simulink model "carpark_shuffler_sim"  (R2025b)
settings: Solver=VariableStepAuto  StartTime=0.0  StopTime=0.06  MaxStep=1e-4  RelTol=1e-4
PreLoadFcn:
  | init_params;
InitFcn:
  | init_params
undefined symbols (not defined in the file or in its folder): LOADP, SENSE, SRC
libraries: fl_lib x63, ee_lib x43, nesl_utility x37
(part 1 of 4)
settings Model: SimulationMode=accelerator  Creator=jazsa  LastModifiedBy=jazsa
settings SolverCC: ZeroCrossAlgorithm=Adaptive
settings DataIOCC: SignalLogging=off

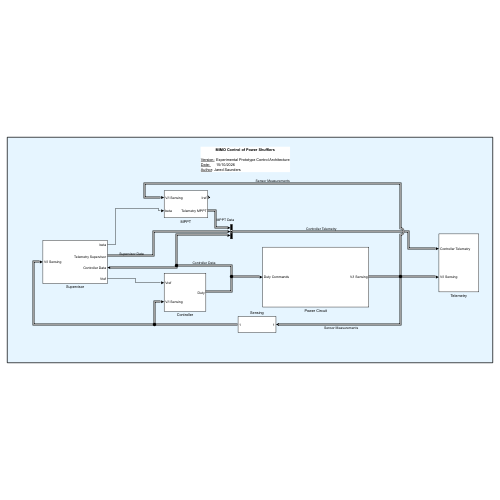
[thumbnail: Simulink's stored preview of the top-level diagram]
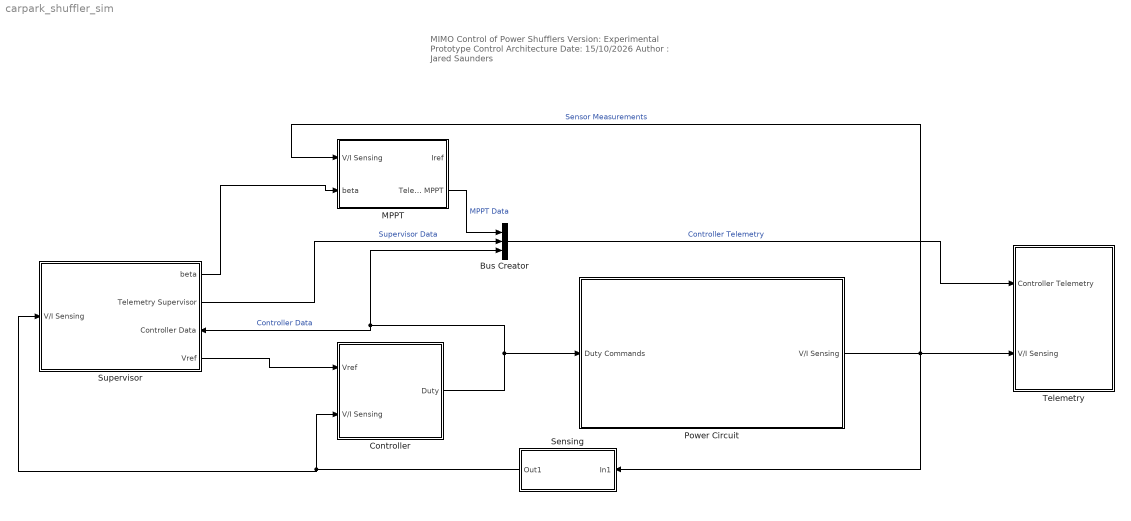
== system carpark_shuffler_sim ==
  note: MIMO Control of Power Shufflers
      |
      | Version: Experimental Prototype Control Architecture
      | Date: 15/10/2026
      | Author : Jared Saunders
  Bus Creator : BusCreator  Inputs=3
  Controller : Subsystem
  MPPT : Subsystem
  Power Circuit : Subsystem
  Sensing : Subsystem
  Supervisor : Subsystem
      settings: PortSchema="{\"entries\":[{\"content\":{\"sides\":[{\"content\":{\"connectorIds\":[\"In1\"]},\"type\":\"ConnectorPlacement.EquallySpacedRectSide\",\"uuid\":\"4149ece3-2139-4a6b-be3b-85e3b5016338\"},{\"content\":{\"connectorIds\":[\"Out1\",\"Out2\",\"In2\",\"Out3\"],\"side\":\"RIGHT\"},\"type\":\"ConnectorPlacement.EquallySpacedRectSide\",\"uuid\":\"a4c8f16e-63c5-4e73-b921-9be0544bd052\"},{\"content\":{\"side\":\"TOP\"},\"type\":\"ConnectorPlacement.EquallySpacedRectSide\",\"uuid\":\"efcb0ad6-b028-42ed-a2aa-71b179d48e39\"}]},\"type\":\"ConnectorPlacement.EquallySpacedConnector\",\"uuid\":\"3400d1fe-81e3-4212-a4bc-db484173b6e0\"}],\"packageUris\":[\"http://schema.mathworks.com/mf0/Connector/R2020b\"],\"version\":\"1.0\"}"
  Telemetry : Subsystem
  wires:
  Supervisor/1(beta) -> MPPT/2(beta)
  Power Circuit/1(V/I Sensing) -> MPPT/1(V/I Sensing), Telemetry/2(V/I Sensing), Sensing/1(In1)  "Sensor Measurements"
  Supervisor/3(Vref) -> Controller/1(Vref)
  Controller/1(Duty) -> Power Circuit/1(Duty Commands), Bus Creator/3, Supervisor/2(Controller Data)  "Controller Data"
  MPPT/2(Telemetry MPPT) -> Bus Creator/1  "MPPT Data"
  Supervisor/2(Telemetry Supervisor) -> Bus Creator/2  "Supervisor Data"
  Bus Creator/1 -> Telemetry/1(Controller Telemetry)  "Controller Telemetry"
  Sensing/1(Out1) -> Supervisor/1(V/I Sensing), Controller/2(V/I Sensing)

== system carpark_shuffler_sim/Controller ==
  Vref : Inport
  V/I Sensing : Inport  Port=2
  Bus Creator : BusCreator  Inputs=4
  Bus Selector : BusSelector  OutputSignals=Module Voltages,Phase Currents
  Controller : MATLAB Function  TreatAsAtomicUnit=on  SystemSampleTime=100e-6
  Demux : Demux
  Duty : Outport
  wires:
  Bus Selector/1 -> Controller/1(VM)  "<Module Voltages>"
  V/I Sensing/1 -> Bus Selector/1
  Bus Selector/2 -> Controller/2(IL)  "<Phase Currents>"
  Vref/1 -> Controller/3(rv)
  Controller/1(d) -> Demux/1
  Demux/1 -> Bus Creator/1  "dA1"
  Demux/2 -> Bus Creator/2  "dB1"
  Demux/3 -> Bus Creator/3  "dA2"
  Demux/4 -> Bus Creator/4  "dB2"
  Bus Creator/1 -> Duty/1

== system carpark_shuffler_sim/MPPT ==
  V/I Sensing : Inport
  beta : Inport  Port=2
  Bus Creator : BusCreator  Inputs=3
  Bus Selector : BusSelector  OutputSignals=String Power Meter
  Bus Selector1 : BusSelector  OutputSignals=V_string,I_string
  Delay : UnitDelay  InitialCondition=12  SampleTime=1e-3  HasFrameUpgradeWarning=on
  Enable : Constant  Value=0
  P&O : MATLAB Function  TreatAsAtomicUnit=on  SystemSampleTime=1e-3
  Iref : Outport
  Telemetry MPPT : Outport  Port=2
  wires:
  beta/1 -> P&O/3(beta)
  V/I Sensing/1 -> Bus Selector/1
  P&O/3(state) -> Bus Creator/3
  Bus Selector1/1 -> P&O/1(Vstr)  "<V_string>"
  Bus Selector1/2 -> P&O/2(Istr)  "<I_string>"
  P&O/1(Iref) -> Bus Creator/1, Delay/1
  Delay/1 -> Iref/1
  Enable/1 -> P&O/4(en)
  Bus Creator/1 -> Telemetry MPPT/1
  P&O/2(Pav) -> Bus Creator/2
  Bus Selector/1 -> Bus Selector1/1  "<String Power Meter>"

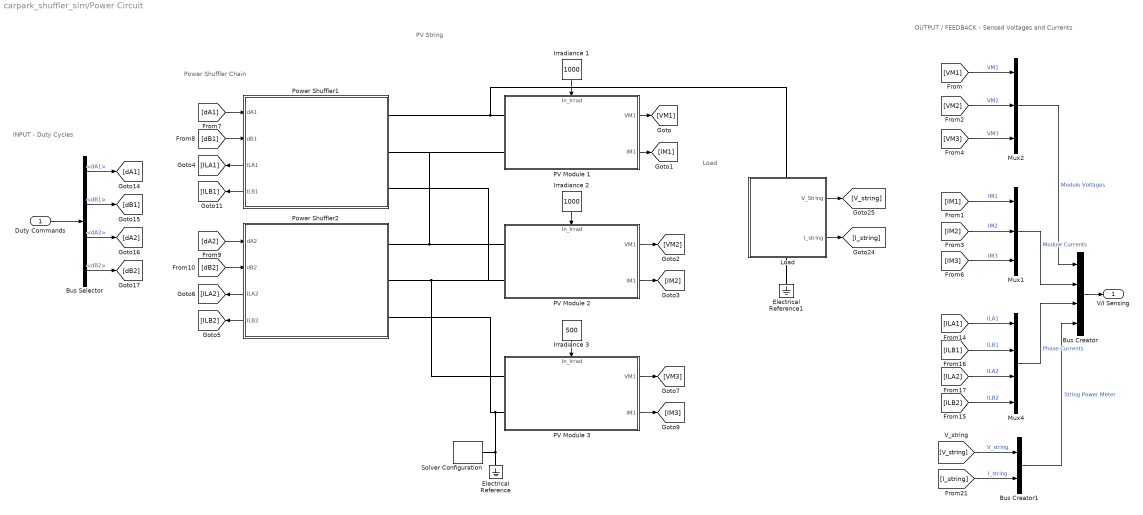
== system carpark_shuffler_sim/Power Circuit ==
  note: OUTPUT / FEEDBACK - Sensed Voltages and Currents
  note: Load
  note: PV String
  note: Power Shuffler Chain
  note: INPUT - Duty Cycles
  Duty Commands : Inport
  Bus Creator : BusCreator  Inputs=4
  Bus Creator1 : BusCreator  Inputs=2
  Bus Selector : BusSelector  OutputSignals=dA1,dB1,dA2,dB2
  Electrical Reference : fl_lib/Electrical/Electrical Elements/Electrical Reference
  Electrical Reference1 : fl_lib/Electrical/Electrical Elements/Electrical Reference
  Irradiance 1 : Constant  Value=1000
  Irradiance 2 : Constant  Value=1000
  Irradiance 3 : Constant  Value=500
  Load : Subsystem
      settings: PortSchema="{\"entries\":[{\"content\":{\"sides\":[{\"content\":{\"connectorIds\":[\"LConn1\"]},\"type\":\"ConnectorPlacement.EquallySpacedRectSide\",\"uuid\":\"6f5f716f-38b7-43f9-a9ba-568c6ccf5920\"},{\"content\":{\"connectorIds\":[\"RConn1\"],\"side\":\"RIGHT\"},\"type\":\"ConnectorPlacement.EquallySpacedRectSide\",\"uuid\":\"74a237b1-90a9-413f-978d-7052f4ba1489\"},{\"content\":{\"side\":\"TOP\"},\"type\":\"ConnectorPlacement.EquallySpacedRectSide\",\"uuid\":\"e5fcb88f-496e-42e0-91fa-e640406c50d5\"},{\"content\":{\"connectorIds\":[\"Out1\",\"Out2\"],\"side\":\"BOTTOM\"},\"type\":\"ConnectorPlacement.EquallySpacedRectSide\",\"uuid\":\"aed6b45d-7ab9-4ae0-b4e0-d20dd58bb9bf\"}]},\"type\":\"ConnectorPlacement.EquallySpacedConnector\",\"uuid\":\"f6ffe9ce-5007-4054-8c52-fa2588b4e46b\"}],\"packageUris\":[\"http://schema.mathworks.com/mf0/Connector/R2020b\"],\"version\":\"1.0\"}"
  Mux1 : Mux  Inputs=3
  Mux2 : Mux  Inputs=3
  Mux4 : Mux
  PV Module 1 : Subsystem
      settings: PortSchema="{\"entries\":[{\"content\":{\"sides\":[{\"content\":{\"connectorIds\":[\"LConn1\",\"LConn2\"]},\"type\":\"ConnectorPlacement.EquallySpacedRectSide\",\"uuid\":\"00bc81be-eb87-4e0d-8cf1-aaf392b111b3\"},{\"content\":{\"connectorIds\":[\"Out1\",\"Out2\"],\"side\":\"RIGHT\"},\"type\":\"ConnectorPlacement.EquallySpacedRectSide\",\"uuid\":\"136cfb59-61d1-4be5-a5a1-62fe670dfe2d\"},{\"content\":{\"connectorIds\":[\"In1\"],\"side\":\"TOP\"},\"type\":\"ConnectorPlacement.EquallySpacedRectSide\",\"uuid\":\"1fa490a3-fddf-446b-98a1-153f2ac018d8\"}]},\"type\":\"ConnectorPlacement.EquallySpacedConnector\",\"uuid\":\"e6ea07bf-3162-47e8-af67-1b2f68d57f24\"}],\"packageUris\":[\"http://schema.mathworks.com/mf0/Connector/R2020b\"],\"version\":\"1.0\"}"
  PV Module 2 : Subsystem
      settings: PortSchema="{\"entries\":[{\"content\":{\"sides\":[{\"content\":{\"connectorIds\":[\"LConn1\",\"LConn2\"]},\"type\":\"ConnectorPlacement.EquallySpacedRectSide\",\"uuid\":\"00bc81be-eb87-4e0d-8cf1-aaf392b111b3\"},{\"content\":{\"connectorIds\":[\"Out1\",\"Out2\"],\"side\":\"RIGHT\"},\"type\":\"ConnectorPlacement.EquallySpacedRectSide\",\"uuid\":\"136cfb59-61d1-4be5-a5a1-62fe670dfe2d\"},{\"content\":{\"connectorIds\":[\"In1\"],\"side\":\"TOP\"},\"type\":\"ConnectorPlacement.EquallySpacedRectSide\",\"uuid\":\"1fa490a3-fddf-446b-98a1-153f2ac018d8\"}]},\"type\":\"ConnectorPlacement.EquallySpacedConnector\",\"uuid\":\"e6ea07bf-3162-47e8-af67-1b2f68d57f24\"}],\"packageUris\":[\"http://schema.mathworks.com/mf0/Connector/R2020b\"],\"version\":\"1.0\"}"
  PV Module 3 : Subsystem
      settings: PortSchema="{\"entries\":[{\"content\":{\"sides\":[{\"content\":{\"connectorIds\":[\"LConn1\",\"LConn2\"]},\"type\":\"ConnectorPlacement.EquallySpacedRectSide\",\"uuid\":\"00bc81be-eb87-4e0d-8cf1-aaf392b111b3\"},{\"content\":{\"connectorIds\":[\"Out1\",\"Out2\"],\"side\":\"RIGHT\"},\"type\":\"ConnectorPlacement.EquallySpacedRectSide\",\"uuid\":\"136cfb59-61d1-4be5-a5a1-62fe670dfe2d\"},{\"content\":{\"connectorIds\":[\"In1\"],\"side\":\"TOP\"},\"type\":\"ConnectorPlacement.EquallySpacedRectSide\",\"uuid\":\"1fa490a3-fddf-446b-98a1-153f2ac018d8\"}]},\"type\":\"ConnectorPlacement.EquallySpacedConnector\",\"uuid\":\"e6ea07bf-3162-47e8-af67-1b2f68d57f24\"}],\"packageUris\":[\"http://schema.mathworks.com/mf0/Connector/R2020b\"],\"version\":\"1.0\"}"
  Power Shuffler1 : Subsystem
      settings: PortSchema="{\"entries\":[{\"content\":{\"sides\":[{\"content\":{\"connectorIds\":[\"LConn1\",\"LConn2\",\"LConn3\"]},\"type\":\"ConnectorPlacement.EquallySpacedRectSide\",\"uuid\":\"00177d11-8382-42fd-b27c-fc09158175e4\"},{\"content\":{\"connectorIds\":[\"In1\",\"In2\",\"Out1\",\"Out2\"],\"side\":\"RIGHT\"},\"type\":\"ConnectorPlacement.EquallySpacedRectSide\",\"uuid\":\"90a306f0-da10-41e1-a725-cfb753adc00c\"},{\"content\":{\"side\":\"TOP\"},\"type\":\"ConnectorPlacement.EquallySpacedRectSide\",\"uuid\":\"612e5683-3ee7-4398-9a5a-0cbdc6c6e41b\"}]},\"type\":\"ConnectorPlacement.EquallySpacedConnector\",\"uuid\":\"1790a0ac-9047-4198-9955-1e7cd181ed81\"}],\"packageUris\":[\"http://schema.mathworks.com/mf0/Connector/R2020b\"],\"version\":\"1.0\"}"
  Power Shuffler2 : Subsystem
      settings: PortSchema="{\"entries\":[{\"content\":{\"sides\":[{\"content\":{\"connectorIds\":[\"LConn1\",\"LConn2\",\"LConn3\"]},\"type\":\"ConnectorPlacement.EquallySpacedRectSide\",\"uuid\":\"00177d11-8382-42fd-b27c-fc09158175e4\"},{\"content\":{\"connectorIds\":[\"In1\",\"In2\",\"Out1\",\"Out2\"],\"side\":\"RIGHT\"},\"type\":\"ConnectorPlacement.EquallySpacedRectSide\",\"uuid\":\"90a306f0-da10-41e1-a725-cfb753adc00c\"},{\"content\":{\"side\":\"TOP\"},\"type\":\"ConnectorPlacement.EquallySpacedRectSide\",\"uuid\":\"612e5683-3ee7-4398-9a5a-0cbdc6c6e41b\"}]},\"type\":\"ConnectorPlacement.EquallySpacedConnector\",\"uuid\":\"1790a0ac-9047-4198-9955-1e7cd181ed81\"}],\"packageUris\":[\"http://schema.mathworks.com/mf0/Connector/R2020b\"],\"version\":\"1.0\"}"
  Solver Configuration : nesl_utility/Solver Configuration  PhysicalDomain=network_engine_domain  SubClassName=solver  LeftPortType=input  RightPortType=generic  Tones=[]  Harmonics=[]  SimulateNoise=off  Profile=off  UseLocalSampling=off  EnableSwitchedLinearOptims=on  FrequencyDomain=off  UseCCode=off  RelTol=0.001  AbsTol=0.001  MinStep=1e-09  ToWorkspace=off  RevertToSquareIcSolve=off  NumHomotopyIterations=100  PhasorMode=off  PhasorModeNumHarmonics=1  ConsistencySolver=NEWTON_XTOL_AFTER_FTOL  IndexReductionMethod=DerivativeReplacement  DoDC=off  ResidualTolerance=1e-09  ConsistencyTolSource=GLOBAL  ConsistencyAbsTol=0.001  ConsistencyRelTol=0.001  ConsistencyTolFactor=0.001  UseLocalSolver=on  LocalSolverChoice=NE_BACKWARD_EULER_ADVANCER  ResolveIndetEquations=on  FunctionEvalNumThread=1  LocalSolverSampleTime=1e-7  DoFixedCost=off  MaxNonlinIter=3  MaxModeIter=2  ComputeImpulses=off  ImpulseIterations=2  LinearAlgebra=auto  LinearAlgebraNumThread=0  EquationFormulation=NE_TIME_EF  DelaysMemoryBudget=1024  AutomaticFiltering=on  FilteringTimeConstant=0.001  PartitionStorageMethod=AS_NEEDED  PartitionMemoryBudget=1024  PartitionMethod=ROBUST  MultibodyUseLocalSolver=off  MultibodyLocalSolverChoice=ODE1  MultibodyLocalSolverSampleTime=0.001
  V/I Sensing : Outport
  wires:
  Load/2(V_String) -> [V_string]
  PV Module 1/1(VM1) -> [VM1]
  Load/1(I_string) -> [I_string]
  Irradiance 3/1 -> PV Module 3/1(In_Irrad)
  Irradiance 2/1 -> PV Module 2/1(In_Irrad)
  Irradiance 1/1 -> PV Module 1/1(In_Irrad)
  Mux2/1 -> Bus Creator/1  "Module Voltages"
  Mux1/1 -> Bus Creator/2  "Module Currents"
  [VM1] -> Mux2/1  "VM1"
  PV Module 1/2(IM1) -> [IM1]
  [IM1] -> Mux1/1  "IM1"
  PV Module 2/1(VM1) -> [VM2]
  [VM2] -> Mux2/2  "VM2"
  PV Module 2/2(IM1) -> [IM2]
  [VM3] -> Mux2/3  "VM3"
  [IM2] -> Mux1/2  "IM2"
  PV Module 3/1(VM1) -> [VM3]
  PV Module 3/2(IM1) -> [IM3]
  [IM3] -> Mux1/3  "IM3"
  Power Shuffler1/1(ILA1) -> [ILA1]
  Power Shuffler1/2(ILB1) -> [ILB1]
  Power Shuffler2/2(ILB2) -> [ILB2]
  Power Shuffler2/1(ILA2) -> [ILA2]
  [ILA1] -> Mux4/1  "ILA1"
  [ILA2] -> Mux4/3  "ILA2"
  [ILB1] -> Mux4/2  "ILB1"
  [ILB2] -> Mux4/4  "ILB2"
  Mux4/1 -> Bus Creator/3  "Phase Currents"
  [dA1] -> Power Shuffler1/1(dA1)
  Duty Commands/1 -> Bus Selector/1
  Bus Selector/1 -> [dA1]  "<dA1>"
  Bus Selector/2 -> [dB1]  "<dB1>"
  [dB1] -> Power Shuffler1/2(dB1)
  [dB2] -> Power Shuffler2/2(dB2)
  [dA2] -> Power Shuffler2/1(dA2)
  Bus Selector/4 -> [dB2]  "<dB2>"
  Bus Selector/3 -> [dA2]  "<dA2>"
  [V_string] -> Bus Creator1/1  "V_string"
  [I_string] -> Bus Creator1/2  "I_string"
  Bus Creator/1 -> V/I Sensing/1
  Bus Creator1/1 -> Bus Creator/4  "String Power Meter"
  connections:
  PV Module 1/LConn2 -- Power Shuffler1/LConn2 -- PV Module 2/LConn1 -- Power Shuffler2/LConn1
  PV Module 1/LConn1 -- Power Shuffler1/LConn1 -- Load/RConn1
  PV Module 2/LConn2 -- Power Shuffler1/LConn3 -- PV Module 3/LConn1 -- Power Shuffler2/LConn2
  Solver Configuration/RConn1 -- PV Module 3/LConn2 -- Power Shuffler2/LConn3 -- Electrical Reference/LConn1
  Electrical Reference1/LConn1 -- Load/LConn1

== system carpark_shuffler_sim/Sensing ==
  In1 : Inport
  Bus Creator : BusCreator  Inputs=4
  Bus Selector : BusSelector  OutputSignals=Module Voltages,Module Currents,Phase Currents,String Power Meter
  Bus Selector1 : BusSelector  OutputSignals=V_string
  Demux : Demux  Outputs=3
  MATLAB Function : MATLAB Function  TreatAsAtomicUnit=on  SystemSampleTime=SENSE.Ts
  To Workspace : ToWorkspace  VariableName=VMm3  SaveFormat=Timeseries  SampleTime=-1
  To Workspace1 : ToWorkspace  VariableName=VMm2  SaveFormat=Timeseries  SampleTime=-1
  To Workspace2 : ToWorkspace  VariableName=VMm1  SaveFormat=Timeseries  SampleTime=-1
  Unit Delay : UnitDelay  InitialCondition=LOADP.Vcv  SampleTime=SENSE.Ts  HasFrameUpgradeWarning=on
  Out1 : Outport
  wires:
  In1/1 -> Bus Selector/1
  Bus Selector/4 -> Bus Selector1/1  "<String Power Meter>"
  Bus Selector/1 -> MATLAB Function/1(VM)  "<Module Voltages>"
  Bus Selector/3 -> MATLAB Function/2(IL)  "<Phase Currents>"
  Bus Selector1/1 -> Unit Delay/1  "<V_string>"
  MATLAB Function/1(VMm) -> Demux/1, Bus Creator/1  "Module Voltages"
  Bus Selector/2 -> Bus Creator/2  "<Module Currents>"
  MATLAB Function/2(ILm) -> Bus Creator/3  "Phase Currents"
  MATLAB Function/3(Vstr_m) -> Bus Creator/4  "Vstr_m"
  Bus Creator/1 -> Out1/1
  Demux/3 -> To Workspace/1
  Demux/2 -> To Workspace1/1
  Demux/1 -> To Workspace2/1
  Unit Delay/1 -> MATLAB Function/3(Vstr)

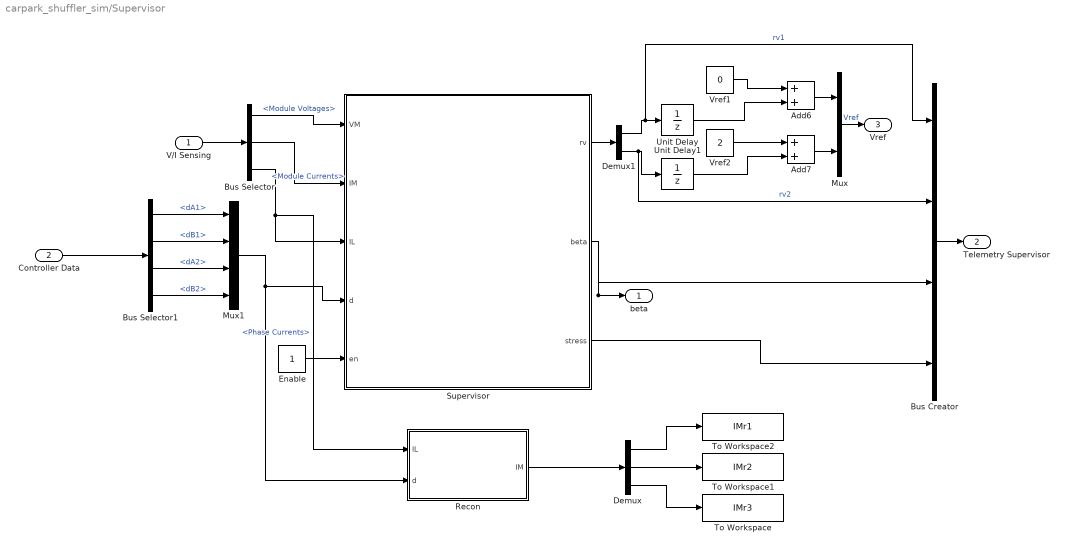
== system carpark_shuffler_sim/Supervisor ==
  V/I Sensing : Inport
  Controller Data : Inport  Port=2
  Add6 : Sum
  Add7 : Sum
  Bus Creator : BusCreator  Inputs=4
  Bus Selector : BusSelector  OutputSignals=Module Voltages,Module Currents,Phase Currents
  Bus Selector1 : BusSelector  OutputSignals=dA1,dB1,dA2,dB2
  Demux : Demux  Outputs=3
  Demux1 : Demux  Outputs=2
  Enable : Constant
  Mux : Mux  Inputs=2
  Mux1 : Mux
  Recon : MATLAB Function  TreatAsAtomicUnit=on
  Supervisor : MATLAB Function  TreatAsAtomicUnit=on  SystemSampleTime=1e-3
  To Workspace : ToWorkspace  VariableName=IMr3  SaveFormat=Timeseries  SampleTime=-1
  To Workspace1 : ToWorkspace  VariableName=IMr2  SaveFormat=Timeseries  SampleTime=-1
  To Workspace2 : ToWorkspace  VariableName=IMr1  SaveFormat=Timeseries  SampleTime=-1
  Unit Delay : UnitDelay  SampleTime=1e-3  HasFrameUpgradeWarning=on
  Unit Delay1 : UnitDelay  SampleTime=1e-3  HasFrameUpgradeWarning=on
  Vref1 : Constant  Value=0
  Vref2 : Constant  Value=2
  beta : Outport
  Telemetry Supervisor : Outport  Port=2
  Vref : Outport  Port=3
  wires:
  Bus Selector/3 -> Recon/1(IL), Supervisor/3(IL)  "<Phase Currents>"
  Bus Creator/1 -> Telemetry Supervisor/1
  Bus Selector1/4 -> Mux1/4  "<dB2>"
  Controller Data/1 -> Bus Selector1/1
  Add6/1 -> Mux/1
  Bus Selector/2 -> Supervisor/2(IM)  "<Module Currents>"
  Vref1/1 -> Add6/1
  Vref2/1 -> Add7/1
  Add7/1 -> Mux/2
  V/I Sensing/1 -> Bus Selector/1
  Enable/1 -> Supervisor/5(en)
  Supervisor/3(stress) -> Bus Creator/4
  Unit Delay1/1 -> Add7/2
  Bus Selector1/1 -> Mux1/1  "<dA1>"
  Bus Selector/1 -> Supervisor/1(VM)  "<Module Voltages>"
  Supervisor/2(beta) -> beta/1, Bus Creator/3
  Mux/1 -> Vref/1  "Vref"
  Bus Selector1/3 -> Mux1/3  "<dA2>"
  Unit Delay/1 -> Add6/2
  Bus Selector1/2 -> Mux1/2  "<dB1>"
  Mux1/1 -> Recon/2(d), Supervisor/4(d)
  Demux/3 -> To Workspace/1
  Demux/2 -> To Workspace1/1
  Demux/1 -> To Workspace2/1
  Recon/1(IM) -> Demux/1
  Supervisor/1(rv) -> Demux1/1
  Demux1/1 -> Bus Creator/1, Unit Delay/1  "rv1"
  Demux1/2 -> Bus Creator/2, Unit Delay1/1  "rv2"

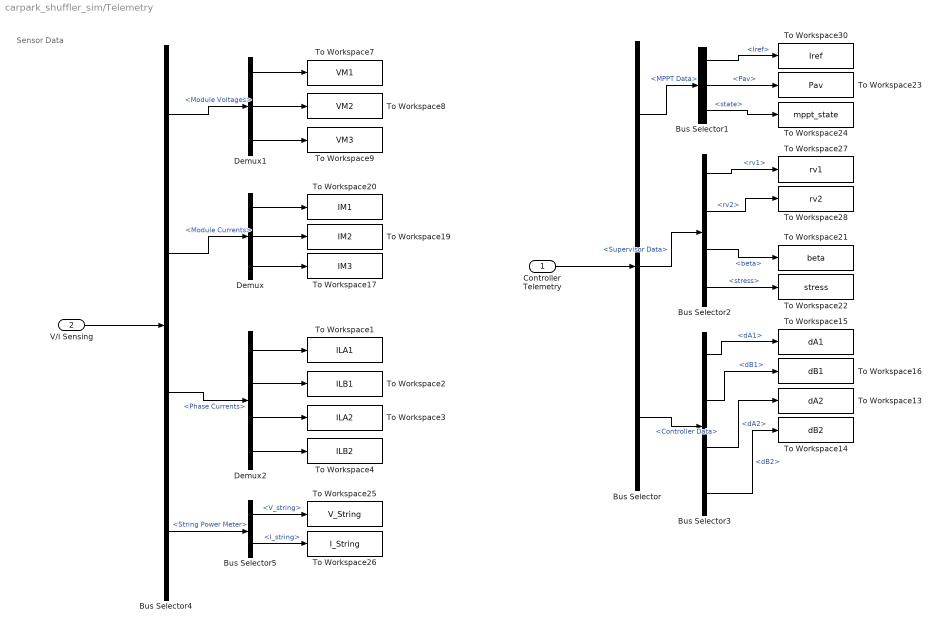
== system carpark_shuffler_sim/Telemetry ==
  note: Sensor Data
  Controller Telemetry : Inport
  V/I Sensing : Inport  Port=2
  Bus Selector : BusSelector  OutputSignals=MPPT Data,Supervisor Data,Controller Data
  Bus Selector1 : BusSelector  OutputSignals=Iref,Pav,state
  Bus Selector2 : BusSelector  OutputSignals=rv1,rv2,beta,stress
  Bus Selector3 : BusSelector  OutputSignals=dA1,dB1,dA2,dB2
  Bus Selector4 : BusSelector  OutputSignals=Module Voltages,Module Currents,Phase Currents,String Power Meter
  Bus Selector5 : BusSelector  OutputSignals=V_string,I_string
  Demux : Demux  Outputs=3
  Demux1 : Demux  Outputs=3
  Demux2 : Demux
  To Workspace1 : ToWorkspace  VariableName=ILA1  SaveFormat=Timeseries  SampleTime=-1
  To Workspace13 : ToWorkspace  VariableName=dA2  SaveFormat=Timeseries  SampleTime=-1
  To Workspace14 : ToWorkspace  VariableName=dB2  SaveFormat=Timeseries  SampleTime=-1
  To Workspace15 : ToWorkspace  VariableName=dA1  SaveFormat=Timeseries  SampleTime=-1
  To Workspace16 : ToWorkspace  VariableName=dB1  SaveFormat=Timeseries  SampleTime=-1
  To Workspace17 : ToWorkspace  VariableName=IM3  SaveFormat=Timeseries  SampleTime=-1
  To Workspace19 : ToWorkspace  VariableName=IM2  SaveFormat=Timeseries  SampleTime=-1
  To Workspace2 : ToWorkspace  VariableName=ILB1  SaveFormat=Timeseries  SampleTime=-1
  To Workspace20 : ToWorkspace  VariableName=IM1  SaveFormat=Timeseries  SampleTime=-1
  To Workspace21 : ToWorkspace  VariableName=beta  SaveFormat=Timeseries  SampleTime=-1
  To Workspace22 : ToWorkspace  VariableName=stress  SaveFormat=Timeseries  SampleTime=-1
  To Workspace23 : ToWorkspace  VariableName=Pav  SaveFormat=Timeseries  SampleTime=-1
  To Workspace24 : ToWorkspace  VariableName=mppt_state  SaveFormat=Timeseries  SampleTime=-1
  To Workspace25 : ToWorkspace  VariableName=V_String  SaveFormat=Timeseries  SampleTime=-1
  To Workspace26 : ToWorkspace  VariableName=I_String  SaveFormat=Timeseries  SampleTime=-1
  To Workspace27 : ToWorkspace  VariableName=rv1  SaveFormat=Timeseries  SampleTime=-1
  To Workspace28 : ToWorkspace  VariableName=rv2  SaveFormat=Timeseries  SampleTime=-1
  To Workspace3 : ToWorkspace  VariableName=ILA2  SaveFormat=Timeseries  SampleTime=-1
  To Workspace30 : ToWorkspace  VariableName=Iref  SaveFormat=Timeseries  SampleTime=-1
  To Workspace4 : ToWorkspace  VariableName=ILB2  SaveFormat=Timeseries  SampleTime=-1
  To Workspace7 : ToWorkspace  VariableName=VM1  SaveFormat=Timeseries  SampleTime=-1
  To Workspace8 : ToWorkspace  VariableName=VM2  SaveFormat=Timeseries  SampleTime=-1
  To Workspace9 : ToWorkspace  VariableName=VM3  SaveFormat=Timeseries  SampleTime=-1
  wires:
  Bus Selector2/2 -> To Workspace28/1  "<rv2>"
  Bus Selector4/3 -> Demux2/1  "<Phase Currents>"
  Demux/1 -> To Workspace20/1
  Demux1/2 -> To Workspace8/1
  Bus Selector/3 -> Bus Selector3/1  "<Controller Data>"
  Bus Selector3/1 -> To Workspace15/1  "<dA1>"
  Demux1/3 -> To Workspace9/1
  Bus Selector/1 -> Bus Selector1/1  "<MPPT Data>"
  Demux2/1 -> To Workspace1/1
  Bus Selector4/2 -> Demux/1  "<Module Currents>"
  Bus Selector5/2 -> To Workspace26/1  "<I_string>"
  Bus Selector2/1 -> To Workspace27/1  "<rv1>"
  Demux2/3 -> To Workspace3/1
  Bus Selector2/3 -> To Workspace21/1  "<beta>"
  Demux2/2 -> To Workspace2/1
  Demux/3 -> To Workspace17/1
  Bus Selector3/3 -> To Workspace13/1  "<dA2>"
  Bus Selector3/2 -> To Workspace16/1  "<dB1>"
  Bus Selector5/1 -> To Workspace25/1  "<V_string>"
  V/I Sensing/1 -> Bus Selector4/1
  Bus Selector4/4 -> Bus Selector5/1  "<String Power Meter>"
  Bus Selector/2 -> Bus Selector2/1  "<Supervisor Data>"
  Controller Telemetry/1 -> Bus Selector/1
  Demux2/4 -> To Workspace4/1
  Bus Selector1/2 -> To Workspace23/1  "<Pav>"
  Demux1/1 -> To Workspace7/1
  Bus Selector1/1 -> To Workspace30/1  "<Iref>"
  Bus Selector2/4 -> To Workspace22/1  "<stress>"
  Bus Selector3/4 -> To Workspace14/1  "<dB2>"
  Bus Selector1/3 -> To Workspace24/1  "<state>"
  Demux/2 -> To Workspace19/1
  Bus Selector4/1 -> Demux1/1  "<Module Voltages>"

== system carpark_shuffler_sim/Power Circuit/Load ==
  Current Sensor : fl_lib/Electrical/Electrical Sensors/Current Sensor
  Load Variant : Subsystem  Variant=on  EmptyChoice=on
  PS-Simulink Converter : nesl_utility/PS-Simulink Converter  PhysicalDomain=network_engine_domain  SubClassName=ps_output  LeftPortType=input  RightPortType=output  PseudoPeriodic=off  Frequencies=[]  VectorFormat=inherit  Unit=inherit  AffineConversion=off
  PS-Simulink Converter1 : nesl_utility/PS-Simulink Converter  PhysicalDomain=network_engine_domain  SubClassName=ps_output  LeftPortType=input  RightPortType=output  PseudoPeriodic=off  Frequencies=[]  VectorFormat=inherit  Unit=inherit  AffineConversion=off
  Voltage Sensor : fl_lib/Electrical/Electrical Sensors/Voltage Sensor
  -ve Terminal : PMIOPort  Side=Left
  +Ve Terminal : PMIOPort  Port=2  Side=Right
  I_string : Outport
  V_String : Outport  Port=2
  wires:
  PS-Simulink Converter/1 -> V_String/1
  PS-Simulink Converter1/1 -> I_string/1
  connections:
  Voltage Sensor/RConn1 -- PS-Simulink Converter/LConn1
  Voltage Sensor/RConn2 -- Current Sensor/RConn2 -- -ve Terminal/RConn1
  Current Sensor/RConn1 -- PS-Simulink Converter1/LConn1
  Voltage Sensor/LConn1 -- +Ve Terminal/RConn1 -- Load Variant/RConn1
  Load Variant/LConn1 -- Current Sensor/LConn1

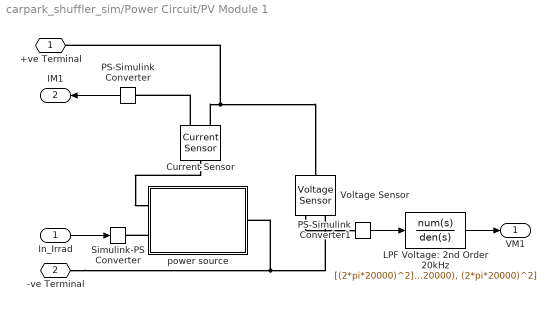
== system carpark_shuffler_sim/Power Circuit/PV Module 1 ==
  In_Irrad : Inport
  Current Sensor : fl_lib/Electrical/Electrical Sensors/Current Sensor
  LPF Voltage: 2nd Order 20kHz : TransferFcn  Numerator=[(2*pi*20000)^2]  Denominator=[1, sqrt(2)*(2*pi*20000), (2*pi*20000)^2]
  PS-Simulink Converter : nesl_utility/PS-Simulink Converter  PhysicalDomain=network_engine_domain  SubClassName=ps_output  LeftPortType=input  RightPortType=output  PseudoPeriodic=off  Frequencies=[]  VectorFormat=inherit  Unit=inherit  AffineConversion=off
  PS-Simulink Converter1 : nesl_utility/PS-Simulink Converter  PhysicalDomain=network_engine_domain  SubClassName=ps_output  LeftPortType=input  RightPortType=output  PseudoPeriodic=off  Frequencies=[]  VectorFormat=inherit  Unit=inherit  AffineConversion=off
  Simulink-PS Converter : nesl_utility/Simulink-PS Converter  PhysicalDomain=network_engine_domain  SubClassName=ps_input  LeftPortType=input  RightPortType=output  PseudoPeriodic=off  Frequencies=[]  NoiseDistribution=none  NoiseParameters=[]  Unit=1  AffineConversion=off  FilteringAndDerivatives=provide  SimscapeFilterOrder=1  InputFilterTimeConstant=0.001  UdotUserProvided=0
  Voltage Sensor : fl_lib/Electrical/Electrical Sensors/Voltage Sensor
  power source : Subsystem  Variant=on  EmptyChoice=on
  +ve Terminal : PMIOPort  Side=Left
  -ve Terminal : PMIOPort  Port=2  Side=Left
  VM1 : Outport
  IM1 : Outport  Port=2
  wires:
  PS-Simulink Converter/1 -> IM1/1
  In_Irrad/1 -> Simulink-PS Converter/1
  PS-Simulink Converter1/1 -> LPF Voltage: 2nd Order 20kHz/1
  LPF Voltage: 2nd Order 20kHz/1 -> VM1/1
  connections:
  Current Sensor/RConn1 -- PS-Simulink Converter/LConn1
  Current Sensor/RConn2 -- Voltage Sensor/LConn1 -- +ve Terminal/RConn1
  Voltage Sensor/RConn1 -- PS-Simulink Converter1/LConn1
  -ve Terminal/RConn1 -- Voltage Sensor/RConn2 -- power source/RConn1
  Current Sensor/LConn1 -- power source/LConn1
  power source/LConn2 -- Simulink-PS Converter/RConn1

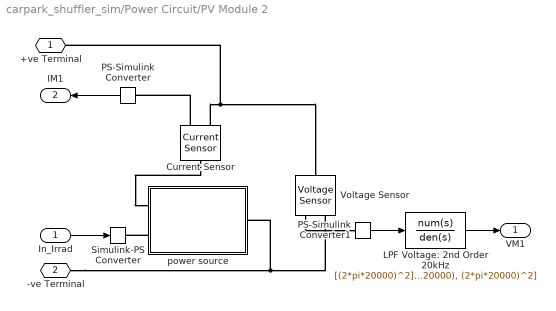
== system carpark_shuffler_sim/Power Circuit/PV Module 2 ==
  In_Irrad : Inport
  Current Sensor : fl_lib/Electrical/Electrical Sensors/Current Sensor
  LPF Voltage: 2nd Order 20kHz : TransferFcn  Numerator=[(2*pi*20000)^2]  Denominator=[1, sqrt(2)*(2*pi*20000), (2*pi*20000)^2]
  PS-Simulink Converter : nesl_utility/PS-Simulink Converter  PhysicalDomain=network_engine_domain  SubClassName=ps_output  LeftPortType=input  RightPortType=output  PseudoPeriodic=off  Frequencies=[]  VectorFormat=inherit  Unit=inherit  AffineConversion=off
  PS-Simulink Converter1 : nesl_utility/PS-Simulink Converter  PhysicalDomain=network_engine_domain  SubClassName=ps_output  LeftPortType=input  RightPortType=output  PseudoPeriodic=off  Frequencies=[]  VectorFormat=inherit  Unit=inherit  AffineConversion=off
  Simulink-PS Converter : nesl_utility/Simulink-PS Converter  PhysicalDomain=network_engine_domain  SubClassName=ps_input  LeftPortType=input  RightPortType=output  PseudoPeriodic=off  Frequencies=[]  NoiseDistribution=none  NoiseParameters=[]  Unit=1  AffineConversion=off  FilteringAndDerivatives=provide  SimscapeFilterOrder=1  InputFilterTimeConstant=0.001  UdotUserProvided=0
  Voltage Sensor : fl_lib/Electrical/Electrical Sensors/Voltage Sensor
  power source : Subsystem  Variant=on  EmptyChoice=on
  +ve Terminal : PMIOPort  Side=Left
  -ve Terminal : PMIOPort  Port=2  Side=Left
  VM1 : Outport
  IM1 : Outport  Port=2
  wires:
  PS-Simulink Converter/1 -> IM1/1
  In_Irrad/1 -> Simulink-PS Converter/1
  PS-Simulink Converter1/1 -> LPF Voltage: 2nd Order 20kHz/1
  LPF Voltage: 2nd Order 20kHz/1 -> VM1/1
  connections:
  Current Sensor/RConn1 -- PS-Simulink Converter/LConn1
  Current Sensor/RConn2 -- Voltage Sensor/LConn1 -- +ve Terminal/RConn1
  Voltage Sensor/RConn1 -- PS-Simulink Converter1/LConn1
  -ve Terminal/RConn1 -- power source/RConn1 -- Voltage Sensor/RConn2
  Current Sensor/LConn1 -- power source/LConn1
  power source/LConn2 -- Simulink-PS Converter/RConn1

== system carpark_shuffler_sim/Power Circuit/PV Module 3 ==
  In_Irrad : Inport
  Current Sensor : fl_lib/Electrical/Electrical Sensors/Current Sensor
  LPF Voltage: 2nd Order 20kHz : TransferFcn  Numerator=[(2*pi*20000)^2]  Denominator=[1, sqrt(2)*(2*pi*20000), (2*pi*20000)^2]
  PS-Simulink Converter : nesl_utility/PS-Simulink Converter  PhysicalDomain=network_engine_domain  SubClassName=ps_output  LeftPortType=input  RightPortType=output  PseudoPeriodic=off  Frequencies=[]  VectorFormat=inherit  Unit=inherit  AffineConversion=off
  PS-Simulink Converter1 : nesl_utility/PS-Simulink Converter  PhysicalDomain=network_engine_domain  SubClassName=ps_output  LeftPortType=input  RightPortType=output  PseudoPeriodic=off  Frequencies=[]  VectorFormat=inherit  Unit=inherit  AffineConversion=off
  Simulink-PS Converter : nesl_utility/Simulink-PS Converter  PhysicalDomain=network_engine_domain  SubClassName=ps_input  LeftPortType=input  RightPortType=output  PseudoPeriodic=off  Frequencies=[]  NoiseDistribution=none  NoiseParameters=[]  Unit=1  AffineConversion=off  FilteringAndDerivatives=provide  SimscapeFilterOrder=1  InputFilterTimeConstant=0.001  UdotUserProvided=0
  Voltage Sensor : fl_lib/Electrical/Electrical Sensors/Voltage Sensor
  power source : Subsystem  Variant=on  EmptyChoice=on
  +ve Terminal : PMIOPort  Side=Left
  -ve Terminal : PMIOPort  Port=2  Side=Left
  VM1 : Outport
  IM1 : Outport  Port=2
  wires:
  PS-Simulink Converter/1 -> IM1/1
  In_Irrad/1 -> Simulink-PS Converter/1
  PS-Simulink Converter1/1 -> LPF Voltage: 2nd Order 20kHz/1
  LPF Voltage: 2nd Order 20kHz/1 -> VM1/1
  connections:
  Current Sensor/RConn1 -- PS-Simulink Converter/LConn1
  Current Sensor/RConn2 -- Voltage Sensor/LConn1 -- +ve Terminal/RConn1
  Voltage Sensor/RConn1 -- PS-Simulink Converter1/LConn1
  -ve Terminal/RConn1 -- power source/RConn1 -- Voltage Sensor/RConn2
  Current Sensor/LConn1 -- power source/LConn1
  power source/LConn2 -- Simulink-PS Converter/RConn1

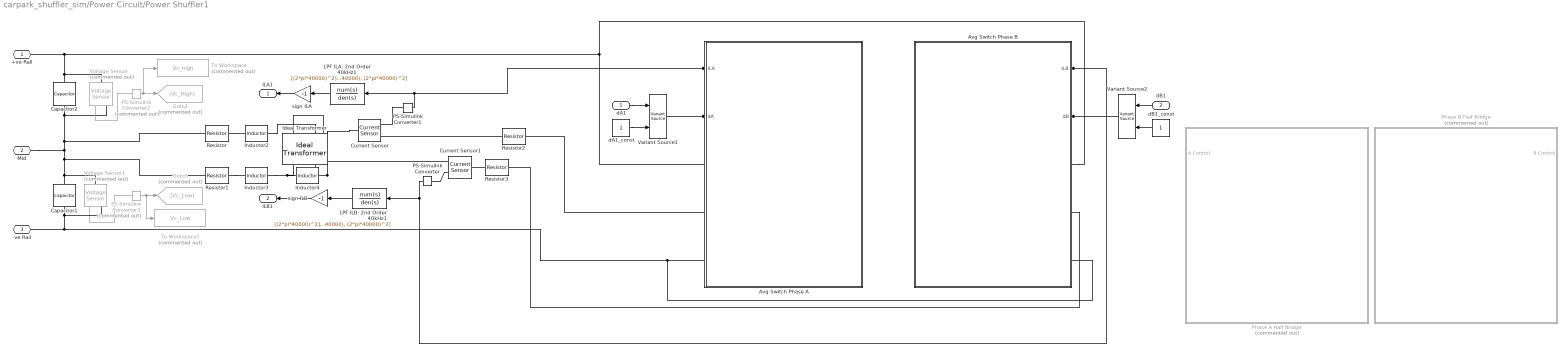
== system carpark_shuffler_sim/Power Circuit/Power Shuffler1 ==
  dA1 : Inport
  dB1 : Inport  Port=2
  Avg Switch Phase A : Subsystem
  Avg Switch Phase B : Subsystem
  Capacitor1 : fl_lib/Electrical/Electrical Elements/Capacitor  c=PLANT.C F  r=PLANT.ESR Ohm  g=0 1/Ohm  i_specify=off  i_priority=None  i=0 A  i_nominal_specify=off  i_nominal_value=1  i_nominal_unit=A  v_specify=off  v_priority=None  v=0 V  v_nominal_specify=off  v_nominal_value=1  v_nominal_unit=V  vc_specify=on  vc_priority=High  vc=LOADP.Vcv/3 V  vc_nominal_specify=off  vc_nominal_value=1  vc_nominal_unit=V
  Capacitor2 : fl_lib/Electrical/Electrical Elements/Capacitor  c=PLANT.C F  r=PLANT.ESR Ohm  g=0 1/Ohm  i_specify=off  i_priority=None  i=0 A  i_nominal_specify=off  i_nominal_value=1  i_nominal_unit=A  v_specify=off  v_priority=None  v=0 V  v_nominal_specify=off  v_nominal_value=1  v_nominal_unit=V  vc_specify=on  vc_priority=High  vc=LOADP.Vcv/3 V  vc_nominal_specify=off  vc_nominal_value=1  vc_nominal_unit=V
  Current Sensor : fl_lib/Electrical/Electrical Sensors/Current Sensor
  Current Sensor1 : fl_lib/Electrical/Electrical Sensors/Current Sensor
  Goto2 : Goto  Commented=on  GotoTag=Vc_High
  Goto3 : Goto  Commented=on  GotoTag=Vc_Low
  Ideal Transformer : fl_lib/Electrical/Electrical Elements/Ideal Transformer  n=1  i1_specify=off  i1_priority=None  i1=0 A  i1_nominal_specify=off  i1_nominal_value=1  i1_nominal_unit=A  v1_specify=off  v1_priority=None  v1=0 V  v1_nominal_specify=off  v1_nominal_value=1  v1_nominal_unit=V  i2_specify=off  i2_priority=None  i2=0 A  i2_nominal_specify=off  i2_nominal_value=1  i2_nominal_unit=A  v2_specify=off  v2_priority=None  v2=0 V  v2_nominal_specify=off  v2_nominal_value=1  v2_nominal_unit=V
  Inductor2 : ee_lib/Passive/Inductor  l=2.05 uH  enable_L_tol=ee.enum.toleranceApplication.none  L_tol=20  tol_distribution=ee.enum.toleranceDistribution.uniform  nSigma=4  r=0 Ohm  g=0 1/Ohm  enable_operating_limits=ee.enum.enable.no  operating_limit_action=ee.enum.passive.reportOpLim.warn  max_working_current=1 A  power_rating=1 W  i_L_specify=off  i_L_priority=High  i_L=0 A  i_L_nominal_specify=off  i_L_nominal_value=1  i_L_nominal_unit=A
  Inductor3 : ee_lib/Passive/Inductor  l=2.05 uH  enable_L_tol=ee.enum.toleranceApplication.none  L_tol=20  tol_distribution=ee.enum.toleranceDistribution.uniform  nSigma=4  r=0 Ohm  g=0 1/Ohm  enable_operating_limits=ee.enum.enable.no  operating_limit_action=ee.enum.passive.reportOpLim.warn  max_working_current=1 A  power_rating=1 W  i_L_specify=off  i_L_priority=High  i_L=0 A  i_L_nominal_specify=off  i_L_nominal_value=1  i_L_nominal_unit=A
  Inductor4 : ee_lib/Passive/Inductor  l=5.85 uH  enable_L_tol=ee.enum.toleranceApplication.none  L_tol=20  tol_distribution=ee.enum.toleranceDistribution.uniform  nSigma=4  r=0 Ohm  g=0 1/Ohm  enable_operating_limits=ee.enum.enable.no  operating_limit_action=ee.enum.passive.reportOpLim.warn  max_working_current=1 A  power_rating=1 W  i_L_specify=off  i_L_priority=High  i_L=0 A  i_L_nominal_specify=off  i_L_nominal_value=1  i_L_nominal_unit=A
  LPF ILA: 2nd Order 40kHz1 : TransferFcn  Numerator=[(2*pi*40000)^2]  Denominator=[1, sqrt(2)*(2*pi*40000), (2*pi*40000)^2]
  LPF ILB: 2nd Order 40kHz1 : TransferFcn  Numerator=[(2*pi*40000)^2]  Denominator=[1, sqrt(2)*(2*pi*40000), (2*pi*40000)^2]
  PS-Simulink Converter : nesl_utility/PS-Simulink Converter  PhysicalDomain=network_engine_domain  SubClassName=ps_output  LeftPortType=input  RightPortType=output  PseudoPeriodic=off  Frequencies=[]  VectorFormat=inherit  Unit=inherit  AffineConversion=off
  PS-Simulink Converter1 : nesl_utility/PS-Simulink Converter  PhysicalDomain=network_engine_domain  SubClassName=ps_output  LeftPortType=input  RightPortType=output  PseudoPeriodic=off  Frequencies=[]  VectorFormat=inherit  Unit=inherit  AffineConversion=off
  PS-Simulink Converter2 : nesl_utility/PS-Simulink Converter  Commented=on  PhysicalDomain=network_engine_domain  SubClassName=ps_output  LeftPortType=input  RightPortType=output  PseudoPeriodic=off  Frequencies=[]  VectorFormat=inherit  Unit=inherit  AffineConversion=off
  PS-Simulink Converter3 : nesl_utility/PS-Simulink Converter  Commented=on  PhysicalDomain=network_engine_domain  SubClassName=ps_output  LeftPortType=input  RightPortType=output  PseudoPeriodic=off  Frequencies=[]  VectorFormat=inherit  Unit=inherit  AffineConversion=off
  Phase A Half Bridge : Subsystem  Commented=on
  Phase B Half Bridge : Subsystem  Commented=on
  Resistor : fl_lib/Electrical/Electrical Elements/Resistor  R=1.85 mOhm  i_specify=off  i_priority=None  i=0 A  i_nominal_specify=off  i_nominal_value=1  i_nominal_unit=A  v_specify=off  v_priority=None  v=0 V  v_nominal_specify=off  v_nominal_value=1  v_nominal_unit=V
  Resistor1 : fl_lib/Electrical/Electrical Elements/Resistor  R=1.85 mOhm  i_specify=off  i_priority=None  i=0 A  i_nominal_specify=off  i_nominal_value=1  i_nominal_unit=A  v_specify=off  v_priority=None  v=0 V  v_nominal_specify=off  v_nominal_value=1  v_nominal_unit=V
  Resistor2 : fl_lib/Electrical/Electrical Elements/Resistor  R=61 mOhm  i_specify=off  i_priority=None  i=0 A  i_nominal_specify=off  i_nominal_value=1  i_nominal_unit=A  v_specify=off  v_priority=None  v=0 V  v_nominal_specify=off  v_nominal_value=1  v_nominal_unit=V
  Resistor3 : fl_lib/Electrical/Electrical Elements/Resistor  R=61 mOhm  i_specify=off  i_priority=None  i=0 A  i_nominal_specify=off  i_nominal_value=1  i_nominal_unit=A  v_specify=off  v_priority=None  v=0 V  v_nominal_specify=off  v_nominal_value=1  v_nominal_unit=V
  To Workspace : ToWorkspace  Commented=on  VariableName=Vc_high  SaveFormat=Timeseries  SampleTime=-1
  To Workspace1 : ToWorkspace  Commented=on  VariableName=Vc_Low  SaveFormat=Timeseries  SampleTime=-1
  Variant Source1 : VariantSource  VariantControls={CTRL_MODE == 1, CTRL_MODE == 0}
  Variant Source2 : VariantSource  VariantControls={CTRL_MODE == 1, CTRL_MODE == 0}
  Voltage Sensor : fl_lib/Electrical/Electrical Sensors/Voltage Sensor  Commented=on
  Voltage Sensor1 : fl_lib/Electrical/Electrical Sensors/Voltage Sensor  Commented=on
  dA1_const : Constant
  dB1_const : Constant
  sign ILA : Gain  Gain=-1
  sign ILB : Gain  Gain=-1
  +ve Rail : PMIOPort  Side=Left
  Mid : PMIOPort  Port=2  Side=Left
  -ve Rail : PMIOPort  Port=3  Side=Left
  ILA1 : Outport
  ILB1 : Outport  Port=2
  wires:
  PS-Simulink Converter1/1 -> Avg Switch Phase A/1(ILA), LPF ILA: 2nd Order 40kHz1/1
  PS-Simulink Converter2/1 -> To Workspace/1, Goto2/1
  PS-Simulink Converter3/1 -> To Workspace1/1, Goto3/1
  PS-Simulink Converter/1 -> Avg Switch Phase B/1(ILB), LPF ILB: 2nd Order 40kHz1/1
  dA1/1 -> Variant Source1/1
  dB1/1 -> Variant Source2/1
  LPF ILA: 2nd Order 40kHz1/1 -> sign ILA/1
  LPF ILB: 2nd Order 40kHz1/1 -> sign ILB/1
  Variant Source1/1 -> Avg Switch Phase A/2(dA)
  dA1_const/1 -> Variant Source1/2
  dB1_const/1 -> Variant Source2/2
  Variant Source2/1 -> Avg Switch Phase B/2(dB)
  sign ILA/1 -> ILA1/1
  sign ILB/1 -> ILB1/1
  connections:
  PS-Simulink Converter1/LConn1 -- Current Sensor/RConn1
  Mid/RConn1 -- Resistor1/LConn1 -- Capacitor1/LConn1 -- Voltage Sensor1/LConn1 -- Resistor/LConn1 -- Capacitor2/RConn1 -- Voltage Sensor/RConn2
  PS-Simulink Converter/LConn1 -- Current Sensor1/RConn1
  Inductor3/RConn1 -- Ideal Transformer/LConn1 -- Inductor4/LConn1
  Ideal Transformer/LConn2 -- Inductor4/RConn1 -- Current Sensor/LConn1
  Inductor2/RConn1 -- Ideal Transformer/RConn2
  Inductor2/LConn1 -- Resistor/RConn1
  Resistor1/RConn1 -- Inductor3/LConn1
  Current Sensor1/RConn2 -- Ideal Transformer/RConn1
  PS-Simulink Converter2/LConn1 -- Voltage Sensor/RConn1
  PS-Simulink Converter3/LConn1 -- Voltage Sensor1/RConn1
  Avg Switch Phase A/LConn3 -- -ve Rail/RConn1 -- Capacitor1/RConn1 -- Voltage Sensor1/RConn2 -- Avg Switch Phase B/LConn3
  Avg Switch Phase A/LConn1 -- Capacitor2/LConn1 -- Voltage Sensor/LConn1 -- +ve Rail/RConn1 -- Avg Switch Phase B/LConn1
  Resistor3/LConn1 -- Current Sensor1/LConn1
  Avg Switch Phase A/LConn2 -- Resistor2/RConn1
  Resistor2/LConn1 -- Current Sensor/RConn2
  Avg Switch Phase B/LConn2 -- Resistor3/RConn1

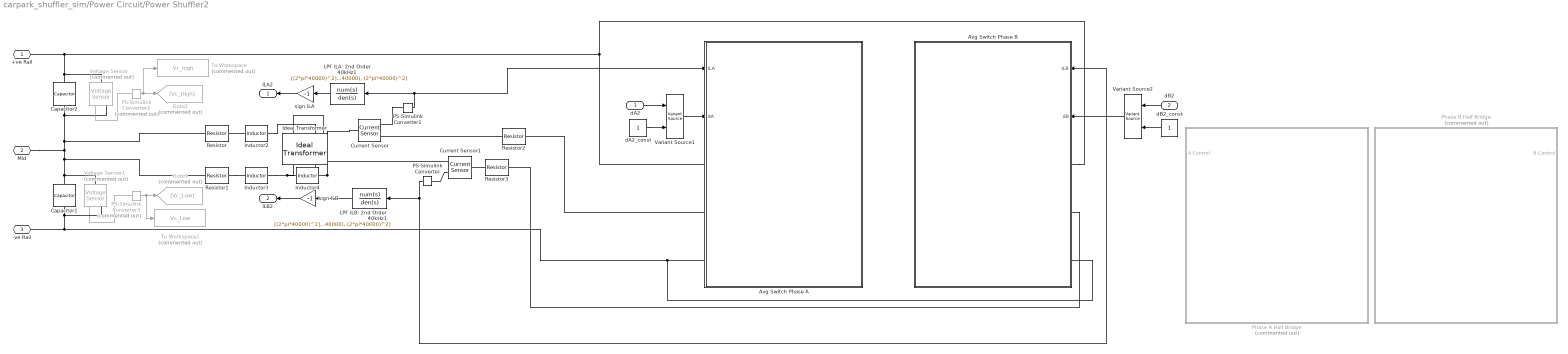
== system carpark_shuffler_sim/Power Circuit/Power Shuffler2 ==
  dA2 : Inport
  dB2 : Inport  Port=2
  Avg Switch Phase A : Subsystem
  Avg Switch Phase B : Subsystem
  Capacitor1 : fl_lib/Electrical/Electrical Elements/Capacitor  c=PLANT.C F  r=PLANT.ESR Ohm  g=0 1/Ohm  i_specify=off  i_priority=None  i=0 A  i_nominal_specify=off  i_nominal_value=1  i_nominal_unit=A  v_specify=off  v_priority=None  v=0 V  v_nominal_specify=off  v_nominal_value=1  v_nominal_unit=V  vc_specify=on  vc_priority=High  vc=LOADP.Vcv/3 V  vc_nominal_specify=off  vc_nominal_value=1  vc_nominal_unit=V
  Capacitor2 : fl_lib/Electrical/Electrical Elements/Capacitor  c=PLANT.C F  r=PLANT.ESR Ohm  g=0 1/Ohm  i_specify=off  i_priority=None  i=0 A  i_nominal_specify=off  i_nominal_value=1  i_nominal_unit=A  v_specify=off  v_priority=None  v=0 V  v_nominal_specify=off  v_nominal_value=1  v_nominal_unit=V  vc_specify=on  vc_priority=High  vc=LOADP.Vcv/3 V  vc_nominal_specify=off  vc_nominal_value=1  vc_nominal_unit=V
  Current Sensor : fl_lib/Electrical/Electrical Sensors/Current Sensor
  Current Sensor1 : fl_lib/Electrical/Electrical Sensors/Current Sensor
  Goto2 : Goto  Commented=on  GotoTag=Vc_High
  Goto3 : Goto  Commented=on  GotoTag=Vc_Low
  Ideal Transformer : fl_lib/Electrical/Electrical Elements/Ideal Transformer  n=1  i1_specify=off  i1_priority=None  i1=0 A  i1_nominal_specify=off  i1_nominal_value=1  i1_nominal_unit=A  v1_specify=off  v1_priority=None  v1=0 V  v1_nominal_specify=off  v1_nominal_value=1  v1_nominal_unit=V  i2_specify=off  i2_priority=None  i2=0 A  i2_nominal_specify=off  i2_nominal_value=1  i2_nominal_unit=A  v2_specify=off  v2_priority=None  v2=0 V  v2_nominal_specify=off  v2_nominal_value=1  v2_nominal_unit=V
  Inductor2 : ee_lib/Passive/Inductor  l=2.05 uH  enable_L_tol=ee.enum.toleranceApplication.none  L_tol=20  tol_distribution=ee.enum.toleranceDistribution.uniform  nSigma=4  r=0 Ohm  g=0 1/Ohm  enable_operating_limits=ee.enum.enable.no  operating_limit_action=ee.enum.passive.reportOpLim.warn  max_working_current=1 A  power_rating=1 W  i_L_specify=off  i_L_priority=High  i_L=0 A  i_L_nominal_specify=off  i_L_nominal_value=1  i_L_nominal_unit=A
  Inductor3 : ee_lib/Passive/Inductor  l=2.05 uH  enable_L_tol=ee.enum.toleranceApplication.none  L_tol=20  tol_distribution=ee.enum.toleranceDistribution.uniform  nSigma=4  r=0 Ohm  g=0 1/Ohm  enable_operating_limits=ee.enum.enable.no  operating_limit_action=ee.enum.passive.reportOpLim.warn  max_working_current=1 A  power_rating=1 W  i_L_specify=off  i_L_priority=High  i_L=0 A  i_L_nominal_specify=off  i_L_nominal_value=1  i_L_nominal_unit=A
  Inductor4 : ee_lib/Passive/Inductor  l=5.85 uH  enable_L_tol=ee.enum.toleranceApplication.none  L_tol=20  tol_distribution=ee.enum.toleranceDistribution.uniform  nSigma=4  r=0 Ohm  g=0 1/Ohm  enable_operating_limits=ee.enum.enable.no  operating_limit_action=ee.enum.passive.reportOpLim.warn  max_working_current=1 A  power_rating=1 W  i_L_specify=off  i_L_priority=High  i_L=0 A  i_L_nominal_specify=off  i_L_nominal_value=1  i_L_nominal_unit=A
  LPF ILA: 2nd Order 40kHz1 : TransferFcn  Numerator=[(2*pi*40000)^2]  Denominator=[1, sqrt(2)*(2*pi*40000), (2*pi*40000)^2]
  LPF ILB: 2nd Order 40kHz1 : TransferFcn  Numerator=[(2*pi*40000)^2]  Denominator=[1, sqrt(2)*(2*pi*40000), (2*pi*40000)^2]
  PS-Simulink Converter : nesl_utility/PS-Simulink Converter  PhysicalDomain=network_engine_domain  SubClassName=ps_output  LeftPortType=input  RightPortType=output  PseudoPeriodic=off  Frequencies=[]  VectorFormat=inherit  Unit=inherit  AffineConversion=off
  PS-Simulink Converter1 : nesl_utility/PS-Simulink Converter  PhysicalDomain=network_engine_domain  SubClassName=ps_output  LeftPortType=input  RightPortType=output  PseudoPeriodic=off  Frequencies=[]  VectorFormat=inherit  Unit=inherit  AffineConversion=off
  PS-Simulink Converter2 : nesl_utility/PS-Simulink Converter  Commented=on  PhysicalDomain=network_engine_domain  SubClassName=ps_output  LeftPortType=input  RightPortType=output  PseudoPeriodic=off  Frequencies=[]  VectorFormat=inherit  Unit=inherit  AffineConversion=off
  PS-Simulink Converter3 : nesl_utility/PS-Simulink Converter  Commented=on  PhysicalDomain=network_engine_domain  SubClassName=ps_output  LeftPortType=input  RightPortType=output  PseudoPeriodic=off  Frequencies=[]  VectorFormat=inherit  Unit=inherit  AffineConversion=off
  Phase A Half Bridge : Subsystem  Commented=on
  Phase B Half Bridge : Subsystem  Commented=on
  Resistor : fl_lib/Electrical/Electrical Elements/Resistor  R=1.85 mOhm  i_specify=off  i_priority=None  i=0 A  i_nominal_specify=off  i_nominal_value=1  i_nominal_unit=A  v_specify=off  v_priority=None  v=0 V  v_nominal_specify=off  v_nominal_value=1  v_nominal_unit=V
  Resistor1 : fl_lib/Electrical/Electrical Elements/Resistor  R=1.85 mOhm  i_specify=off  i_priority=None  i=0 A  i_nominal_specify=off  i_nominal_value=1  i_nominal_unit=A  v_specify=off  v_priority=None  v=0 V  v_nominal_specify=off  v_nominal_value=1  v_nominal_unit=V
  Resistor2 : fl_lib/Electrical/Electrical Elements/Resistor  R=61 mOhm  i_specify=off  i_priority=None  i=0 A  i_nominal_specify=off  i_nominal_value=1  i_nominal_unit=A  v_specify=off  v_priority=None  v=0 V  v_nominal_specify=off  v_nominal_value=1  v_nominal_unit=V
  Resistor3 : fl_lib/Electrical/Electrical Elements/Resistor  R=61 mOhm  i_specify=off  i_priority=None  i=0 A  i_nominal_specify=off  i_nominal_value=1  i_nominal_unit=A  v_specify=off  v_priority=None  v=0 V  v_nominal_specify=off  v_nominal_value=1  v_nominal_unit=V
  To Workspace : ToWorkspace  Commented=on  VariableName=Vc_high  SaveFormat=Timeseries  SampleTime=-1
  To Workspace1 : ToWorkspace  Commented=on  VariableName=Vc_Low  SaveFormat=Timeseries  SampleTime=-1
  Variant Source1 : VariantSource  VariantControls={CTRL_MODE == 1, CTRL_MODE == 0}
  Variant Source2 : VariantSource  VariantControls={CTRL_MODE == 1, CTRL_MODE == 0}
  Voltage Sensor : fl_lib/Electrical/Electrical Sensors/Voltage Sensor  Commented=on
  Voltage Sensor1 : fl_lib/Electrical/Electrical Sensors/Voltage Sensor  Commented=on
  dA2_const : Constant
  dB2_const : Constant
  sign ILA : Gain  Gain=-1
  sign ILB : Gain  Gain=-1
  +ve Rail : PMIOPort  Side=Left
  Mid : PMIOPort  Port=2  Side=Left
  -ve Rail : PMIOPort  Port=3  Side=Left
  ILA2 : Outport
  ILB2 : Outport  Port=2
  wires:
  PS-Simulink Converter1/1 -> Avg Switch Phase A/1(ILA), LPF ILA: 2nd Order 40kHz1/1
  PS-Simulink Converter2/1 -> To Workspace/1, Goto2/1
  PS-Simulink Converter3/1 -> To Workspace1/1, Goto3/1
  PS-Simulink Converter/1 -> Avg Switch Phase B/1(ILB), LPF ILB: 2nd Order 40kHz1/1
  dA2/1 -> Variant Source1/1
  dB2/1 -> Variant Source2/1
  LPF ILA: 2nd Order 40kHz1/1 -> sign ILA/1
  LPF ILB: 2nd Order 40kHz1/1 -> sign ILB/1
  dA2_const/1 -> Variant Source1/2
  Variant Source1/1 -> Avg Switch Phase A/2(dA)
  dB2_const/1 -> Variant Source2/2
  Variant Source2/1 -> Avg Switch Phase B/2(dB)
  sign ILB/1 -> ILB2/1
  sign ILA/1 -> ILA2/1
  connections:
  PS-Simulink Converter1/LConn1 -- Current Sensor/RConn1
  Mid/RConn1 -- Resistor1/LConn1 -- Capacitor1/LConn1 -- Voltage Sensor1/LConn1 -- Resistor/LConn1 -- Capacitor2/RConn1 -- Voltage Sensor/RConn2
  PS-Simulink Converter/LConn1 -- Current Sensor1/RConn1
  Inductor3/RConn1 -- Ideal Transformer/LConn1 -- Inductor4/LConn1
  Ideal Transformer/LConn2 -- Inductor4/RConn1 -- Current Sensor/LConn1
  Inductor2/RConn1 -- Ideal Transformer/RConn2
  Inductor2/LConn1 -- Resistor/RConn1
  Resistor1/RConn1 -- Inductor3/LConn1
  Current Sensor1/RConn2 -- Ideal Transformer/RConn1
  PS-Simulink Converter2/LConn1 -- Voltage Sensor/RConn1
  PS-Simulink Converter3/LConn1 -- Voltage Sensor1/RConn1
  Avg Switch Phase A/LConn3 -- -ve Rail/RConn1 -- Capacitor1/RConn1 -- Voltage Sensor1/RConn2 -- Avg Switch Phase B/LConn3
  Avg Switch Phase A/LConn1 -- Capacitor2/LConn1 -- Voltage Sensor/LConn1 -- +ve Rail/RConn1 -- Avg Switch Phase B/LConn1
  Resistor3/LConn1 -- Current Sensor1/LConn1
  Avg Switch Phase A/LConn2 -- Resistor2/RConn1
  Resistor2/LConn1 -- Current Sensor/RConn2
  Avg Switch Phase B/LConn2 -- Resistor3/RConn1

== system carpark_shuffler_sim/Power Circuit/Load/Load Variant ==
  CC : Subsystem  VariantControl=LOAD_ID == 1
  CV : Subsystem  VariantControl=LOAD_ID == 2
  +ve : PMIOPort  Side=Right
  -ve : PMIOPort  Port=2  Side=Left

== system carpark_shuffler_sim/Power Circuit/PV Module 1/power source ==
  BENCH : Subsystem  VariantControl=SETUP_ID == 1
  PV80 : Subsystem  VariantControl=SETUP_ID == 2
  +ve : PMIOPort  Side=Left
  Irrad : PMIOPort  Port=2  Side=Left
  -ve : PMIOPort  Port=3  Side=Right

== system carpark_shuffler_sim/Power Circuit/PV Module 2/power source ==
  BENCH : Subsystem  VariantControl=SETUP_ID == 1
  PV80 : Subsystem  VariantControl=SETUP_ID == 2
  +ve : PMIOPort  Side=Left
  Irrad : PMIOPort  Port=2  Side=Left
  -ve : PMIOPort  Port=3  Side=Right

== system carpark_shuffler_sim/Power Circuit/PV Module 3/power source ==
  BENCH : Subsystem  VariantControl=SETUP_ID == 1
  PV80 : Subsystem  VariantControl=SETUP_ID == 2
  +ve : PMIOPort  Side=Left
  Irrad : PMIOPort  Port=2  Side=Left
  -ve : PMIOPort  Port=3  Side=Right

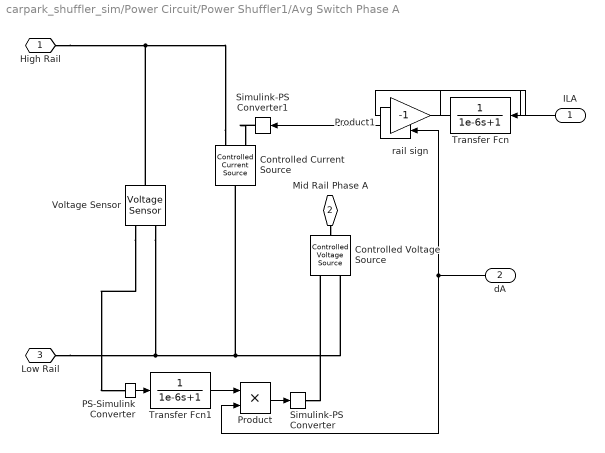
== system carpark_shuffler_sim/Power Circuit/Power Shuffler1/Avg Switch Phase A ==
  ILA : Inport
  dA : Inport  Port=2
  Controlled Current Source : fl_lib/Electrical/Electrical Sources/Controlled Current Source
  Controlled Voltage Source : fl_lib/Electrical/Electrical Sources/Controlled Voltage Source
  PS-Simulink Converter : nesl_utility/PS-Simulink Converter  PhysicalDomain=network_engine_domain  SubClassName=ps_output  LeftPortType=input  RightPortType=output  PseudoPeriodic=off  Frequencies=[]  VectorFormat=inherit  Unit=inherit  AffineConversion=off
  Product : Product
  Product1 : Product
  Simulink-PS Converter : nesl_utility/Simulink-PS Converter  PhysicalDomain=network_engine_domain  SubClassName=ps_input  LeftPortType=input  RightPortType=output  PseudoPeriodic=off  Frequencies=[]  NoiseDistribution=none  NoiseParameters=[]  Unit=1  AffineConversion=off  FilteringAndDerivatives=provide  SimscapeFilterOrder=1  InputFilterTimeConstant=0.001  UdotUserProvided=0
  Simulink-PS Converter1 : nesl_utility/Simulink-PS Converter  PhysicalDomain=network_engine_domain  SubClassName=ps_input  LeftPortType=input  RightPortType=output  PseudoPeriodic=off  Frequencies=[]  NoiseDistribution=none  NoiseParameters=[]  Unit=1  AffineConversion=off  FilteringAndDerivatives=provide  SimscapeFilterOrder=1  InputFilterTimeConstant=0.001  UdotUserProvided=0
  Transfer Fcn : TransferFcn  Denominator=[1e-6 1]
  Transfer Fcn1 : TransferFcn  Denominator=[1e-6 1]
  Voltage Sensor : fl_lib/Electrical/Electrical Sensors/Voltage Sensor
  rail sign : Gain  Gain=-1
      settings: AttributesFormatString=Sensor A reads the current INTO the switch node (sensor B reads OUT); the rail current source needs OUT. Energy balance check 15 Oct.
  High Rail : PMIOPort  Side=Left
  Mid Rail Phase A : PMIOPort  Port=2  Side=Left
  Low Rail : PMIOPort  Port=3  Side=Left
  wires:
  PS-Simulink Converter/1 -> Transfer Fcn1/1
  Transfer Fcn1/1 -> Product/1
  Product1/1 -> Simulink-PS Converter1/1
  dA/1 -> Product1/2, Product/2
  Transfer Fcn/1 -> Product1/1
  Product/1 -> Simulink-PS Converter/1
  ILA/1 -> rail sign/1
  rail sign/1 -> Transfer Fcn/1
  connections:
  Controlled Voltage Source/RConn2 -- Controlled Current Source/LConn1 -- Low Rail/RConn1 -- Voltage Sensor/RConn2
  Controlled Current Source/RConn2 -- High Rail/RConn1 -- Voltage Sensor/LConn1
  Simulink-PS Converter/RConn1 -- Controlled Voltage Source/RConn1
  Mid Rail Phase A/RConn1 -- Controlled Voltage Source/LConn1
  Voltage Sensor/RConn1 -- PS-Simulink Converter/LConn1
  Simulink-PS Converter1/RConn1 -- Controlled Current Source/RConn1

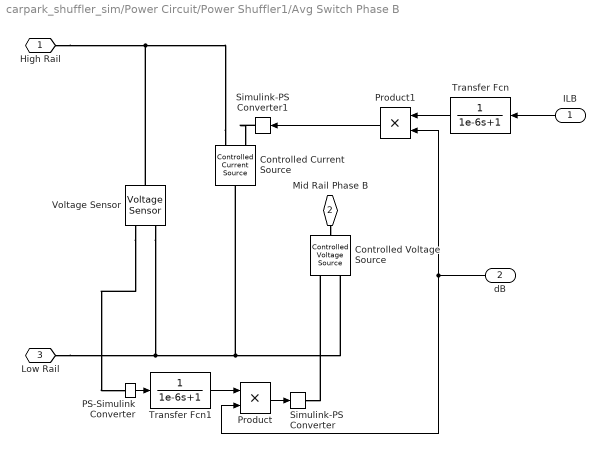
== system carpark_shuffler_sim/Power Circuit/Power Shuffler1/Avg Switch Phase B ==
  ILB : Inport
  dB : Inport  Port=2
  Controlled Current Source : fl_lib/Electrical/Electrical Sources/Controlled Current Source
  Controlled Voltage Source : fl_lib/Electrical/Electrical Sources/Controlled Voltage Source
  PS-Simulink Converter : nesl_utility/PS-Simulink Converter  PhysicalDomain=network_engine_domain  SubClassName=ps_output  LeftPortType=input  RightPortType=output  PseudoPeriodic=off  Frequencies=[]  VectorFormat=inherit  Unit=inherit  AffineConversion=off
  Product : Product
  Product1 : Product
  Simulink-PS Converter : nesl_utility/Simulink-PS Converter  PhysicalDomain=network_engine_domain  SubClassName=ps_input  LeftPortType=input  RightPortType=output  PseudoPeriodic=off  Frequencies=[]  NoiseDistribution=none  NoiseParameters=[]  Unit=1  AffineConversion=off  FilteringAndDerivatives=provide  SimscapeFilterOrder=1  InputFilterTimeConstant=0.001  UdotUserProvided=0
  Simulink-PS Converter1 : nesl_utility/Simulink-PS Converter  PhysicalDomain=network_engine_domain  SubClassName=ps_input  LeftPortType=input  RightPortType=output  PseudoPeriodic=off  Frequencies=[]  NoiseDistribution=none  NoiseParameters=[]  Unit=1  AffineConversion=off  FilteringAndDerivatives=provide  SimscapeFilterOrder=1  InputFilterTimeConstant=0.001  UdotUserProvided=0
  Transfer Fcn : TransferFcn  Denominator=[1e-6 1]
  Transfer Fcn1 : TransferFcn  Denominator=[1e-6 1]
  Voltage Sensor : fl_lib/Electrical/Electrical Sensors/Voltage Sensor
  High Rail : PMIOPort  Side=Left
  Mid Rail Phase B : PMIOPort  Port=2  Side=Left
  Low Rail : PMIOPort  Port=3  Side=Left
  wires:
  PS-Simulink Converter/1 -> Transfer Fcn1/1
  Transfer Fcn1/1 -> Product/1
  Product1/1 -> Simulink-PS Converter1/1
  dB/1 -> Product1/2, Product/2
  Transfer Fcn/1 -> Product1/1
  ILB/1 -> Transfer Fcn/1
  Product/1 -> Simulink-PS Converter/1
  connections:
  Controlled Voltage Source/RConn2 -- Controlled Current Source/LConn1 -- Low Rail/RConn1 -- Voltage Sensor/RConn2
  Controlled Current Source/RConn2 -- High Rail/RConn1 -- Voltage Sensor/LConn1
  Simulink-PS Converter/RConn1 -- Controlled Voltage Source/RConn1
  Mid Rail Phase B/RConn1 -- Controlled Voltage Source/LConn1
  Voltage Sensor/RConn1 -- PS-Simulink Converter/LConn1
  Simulink-PS Converter1/RConn1 -- Controlled Current Source/RConn1
